simulink model "BO_diag"  (R2024b)
settings: Solver=VariableStepAuto  StartTime=0.0  StopTime=10.0  RelTol=1e-3
undefined symbols (not defined in the file): plant_ss_diag
settings Model: Creator=dsagn  LastModifiedBy=dsagn
settings ConfigComp: CovMetricSettings=de  CovBoundaryAbsTol=1.0e-5

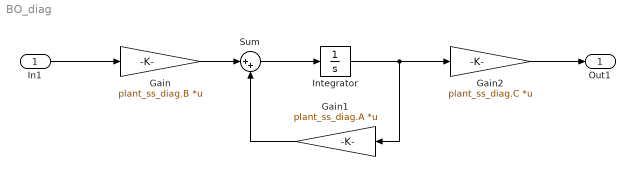
== system BO_diag ==
  In1 : Inport
  Gain : Gain  Gain=plant_ss_diag.B  Multiplication=Matrix(K*u) (u vector)
  Gain1 : Gain  Gain=plant_ss_diag.A  Multiplication=Matrix(K*u) (u vector)
  Gain2 : Gain  Gain=plant_ss_diag.C  Multiplication=Matrix(K*u) (u vector)
  Integrator : Integrator
  Sum : Sum  Inputs=|++
  Out1 : Outport
  wires:
  Sum/1 -> Integrator/1
  Integrator/1 -> Gain1/1, Gain2/1
  Gain1/1 -> Sum/2
  Gain/1 -> Sum/1
  In1/1 -> Gain/1
  Gain2/1 -> Out1/1
